simulink library "probeLib"  (Simulink 10.3)
settings: Solver=VariableStepAuto  StartTime=0.0  StopTime=10.0  RelTol=1e-3
libraries: simulink x1
Description:
  | Library description
settings Model: Creator=matlabdomain  ModifiedByFormat=matlabdomain  LastModifiedBy=matlabdomain

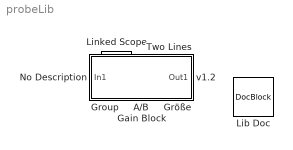
== system probeLib ==
  A/B : Subsystem  mask(SlashType){gain=2, mode=fast, flag=on}
      mask prompts: gain "Gain value"; flag "Enable"
      mask help: Name has a slash.
      mask TypeOptions mode: fast | slow
  Gain Block : Subsystem  mask(GainType){gain=2, mode=fast, flag=on}
      mask prompts: gain "Gain value"; flag "Enable"
      mask help: Top masked block description.
      mask Help: Top masked help.
      mask TypeOptions mode: fast | slow
  Group : Subsystem  Description=Unmasked group description
  Größe : Subsystem  mask(UnicodeType){gain=2, mode=fast, flag=on}
      mask prompts: gain "Gain value"; flag "Enable"
      mask help: Name is non-ASCII: Größe.
      mask TypeOptions mode: fast | slow
  Lib Doc : simulink/Model-Wide Utilities/DocBlock  DocumentType=Text
      content=|
      | Library DocBlock text.
  Linked Scope : Scope
  No Description : Subsystem  mask{gain=2, mode=fast, flag=on}
      mask prompts: gain "Gain value"; flag "Enable"
      mask TypeOptions mode: fast | slow
  Two Lines : Subsystem  mask(NewlineType){gain=2, mode=fast, flag=on}
      mask prompts: gain "Gain value"; flag "Enable"
      mask help: Name has a newline.
      mask TypeOptions mode: fast | slow
  v1.2 : Subsystem  mask(DotType){gain=2, mode=fast, flag=on}
      mask prompts: gain "Gain value"; flag "Enable"
      mask help: Name has a dot.
      mask TypeOptions mode: fast | slow

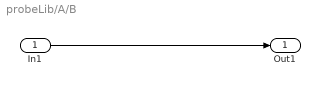
== system probeLib/A/B ==
  In1 : Inport
  Out1 : Outport
  wires:
  In1/1 -> Out1/1

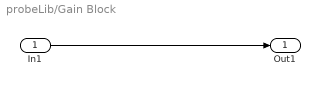
== system probeLib/Gain Block ==
  In1 : Inport
  Out1 : Outport
  wires:
  In1/1 -> Out1/1

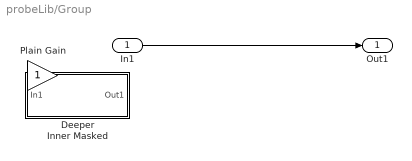
== system probeLib/Group ==
  In1 : Inport
  Deeper : Subsystem
  Inner Masked : Subsystem  mask(InnerType){gain=2, mode=fast, flag=on}
      mask prompts: gain "Gain value"; flag "Enable"
      mask help: Inner masked description.
      mask Help: Inner help.
      mask TypeOptions mode: fast | slow
  Plain Gain : Gain
  Out1 : Outport
  wires:
  In1/1 -> Out1/1

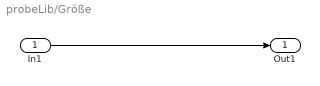
== system probeLib/Größe ==
  In1 : Inport
  Out1 : Outport
  wires:
  In1/1 -> Out1/1

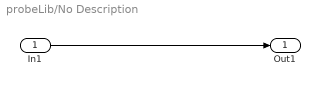
== system probeLib/No Description ==
  In1 : Inport
  Out1 : Outport
  wires:
  In1/1 -> Out1/1

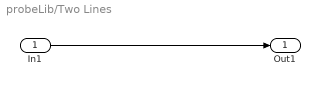
== system probeLib/Two Lines ==
  In1 : Inport
  Out1 : Outport
  wires:
  In1/1 -> Out1/1

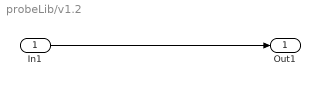
== system probeLib/v1.2 ==
  In1 : Inport
  Out1 : Outport
  wires:
  In1/1 -> Out1/1

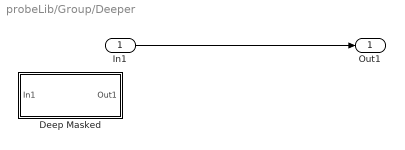
== system probeLib/Group/Deeper ==
  In1 : Inport
  Deep Masked : Subsystem  mask(DeepType){gain=2, mode=fast, flag=on}
      mask prompts: gain "Gain value"; flag "Enable"
      mask help: Deep masked description.
      mask TypeOptions mode: fast | slow
  Out1 : Outport
  wires:
  In1/1 -> Out1/1

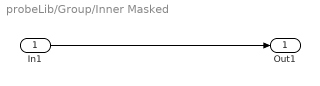
== system probeLib/Group/Inner Masked ==
  In1 : Inport
  Out1 : Outport
  wires:
  In1/1 -> Out1/1

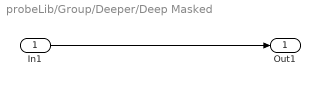
== system probeLib/Group/Deeper/Deep Masked ==
  In1 : Inport
  Out1 : Outport
  wires:
  In1/1 -> Out1/1
